simulink model "sys1"  (R2023b)
settings: Solver=VariableStepAuto  StartTime=0.0  StopTime=30e-3  RelTol=1e-3
InitFcn:
  | fs = 100e6;
  | ts = 1 / fs;
values from neighbouring files (symbols this model uses):
  c = 3e8    (= 300000000)    [init_param.m]
  H_az1 = zeros(numSamples,numPulses)    [init_param.m]
  H_az2 = zeros(numSamples,numPulses)    [init_param.m]
  H_ref = fft(conj(fliplr(txChirp)), numSamples)    [init_param.m]
  rawData = rawData + 0.01 * (randn(size(rawData)) + 1j * randn(size(rawData)))    [init_param.m]
  x1 = zeros(size(rawData))    [main.m]
  x2 = zeros(size(x1))    [main.m]
  x3 = zeros(size(x2))    [main.m]
  x4 = zeros(size(x3))    [main.m]
  x5 = zeros(size(x4))    [main.m]
  x6 = zeros(size(x5))    [main.m]
  xx4 = zeros(size(xx3))    [main.m]
  xx5 = zeros(size(xx4))    [main.m]
  xx6 = zeros(size(xx5))    [main.m]
undefined symbols (not defined in the file or in its folder): ffva1156, w2, w3, w4, w5, w6, w7, w8, w9, ww2, ww3, ww4, ww5, ww6, ww7, ww8, ww9, xcku095
libraries: hdlBasic x917, hdlDSPIP x18, dspsrcs4 x12, vmcUtilities x1
(part 1 of 9)
settings Model: Creator=abbas  LastModifiedBy=87544

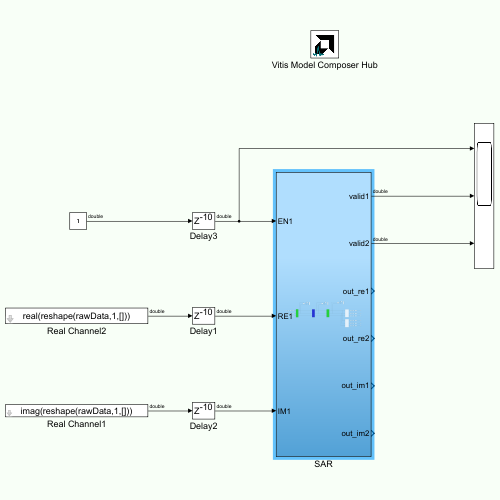
[thumbnail: Simulink's stored preview of the top-level diagram]
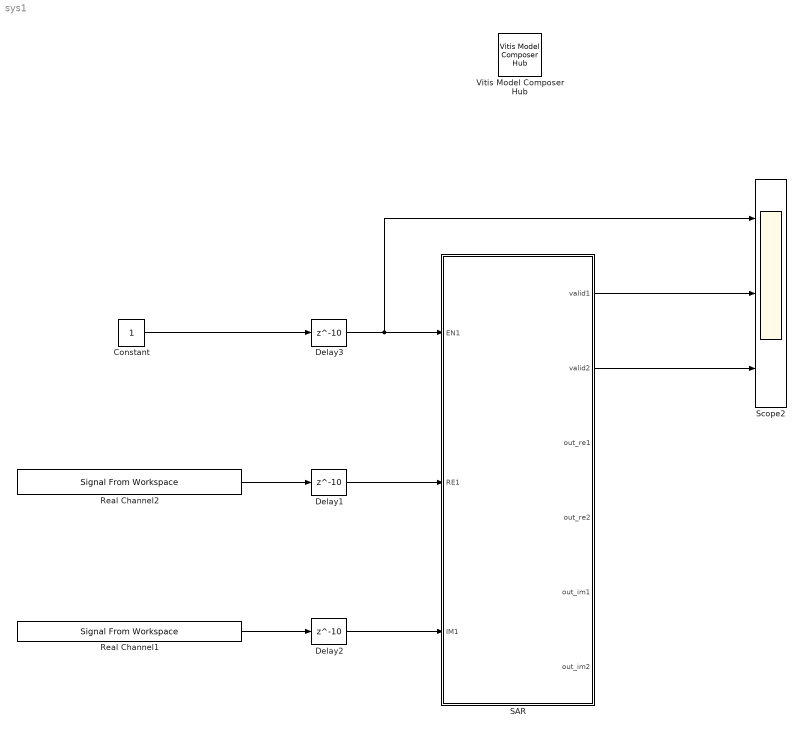
== system sys1 ==
  Constant : Constant
  Delay1 : Delay  DelayLength=10  InitialCondition=0  UseCircularBuffer=on
  Delay2 : Delay  DelayLength=10  InitialCondition=0  UseCircularBuffer=on
  Delay3 : Delay  DelayLength=10  InitialCondition=0  UseCircularBuffer=on
  Real Channel1 : dspsrcs4/Signal From Workspace  X=imag(reshape(rawData,1,[]))  Ts=ts  nsamps=1  OutputAfterFinalValue=Cyclic repetition  ignoreOrWarnInputAndFrameLengths=off  OutputFrames=on
  Real Channel2 : dspsrcs4/Signal From Workspace  X=real(reshape(rawData,1,[]))  Ts=ts  nsamps=1  OutputAfterFinalValue=Cyclic repetition  ignoreOrWarnInputAndFrameLengths=off  OutputFrames=on
  SAR : Subsystem
  Scope2 : Scope  NumInputPorts=3
  Vitis Model Composer Hub : vmcUtilities/Vitis Model Composer Hub  Tag=genX  CodeGeneration=off  SubsystemName=sar_sys8  TargetDirectory=./code  ExportType=System Generator  IpVendor=xilinx.com  IpLibrary=hls  IpVersion=1.0  IpHWLanguage=Verilog  AieCompilerOptions={}  AieSimulatorOptions={}  CreateTestbench=off  TestbenchStackSize=10  RunRtlSim=off  RunCSim=off  RunAieSim=off  AieSimTimeout=50000  RunAieSimProfiling=off  LaunchVitisAnalyzer=off  PlotOutput=off  RunX86Sim=off  X86SimTimeout=10  GenHwImage=off  GenLibadfXo=off  PlatformType=Not Specified  HwSystemType=Baremetal  HwValidationTarget=hw  ProjDevice=xcku095-ffva1156-1-c  ProjDevicePart=xcku095-ffva1156-1-c  AIEType=None  SamplePeriod=-1  ClockFrequency=200  DataPathParallelism=1  xilinxfamily=kintexu  part=xcku095  speed=-1-c  package=ffva1156  directory=C:/Users/87544/Desktop/Low-Latency SAR Processing/mat/netlist\ip\sar_sys8\src  testbench=off  incr_netlist=off  synthesis_tool=Vivado  clock_wrapper=Clock Enables  dbl_ovrd=According to Block Masks  dcm_input_clock_period=10  sysclk_period=10  simulink_period=10e-9  eval_field=0  IPInfoJsonString="{\"HDLSubsystem\":{\"SubsystemName\":\"SAR\",\"IPName\":\"SAR\",\"IPLibrary\":\"VMC\",\"IPVendor\":\"User Company\",\"IPVersion\":\"1.0\",\"TargetDirectory\":\"C:/Users/87544/Desktop/SAR/netlist\",\"SubsystemDir\":\"C:/Users/87544/Desktop/SAR/netlist\\\\ip\\\\SAR\"}}"  LogFileName=''  NThreads=4
  wires:
  Delay3/1 -> Scope2/1, SAR/1(EN1)
  Real Channel2/1 -> Delay1/1
  Constant/1 -> Delay3/1
  Delay2/1 -> SAR/3(IM1)
  Real Channel1/1 -> Delay2/1
  Delay1/1 -> SAR/2(RE1)
  SAR/1(valid1) -> Scope2/2
  SAR/2(valid2) -> Scope2/3

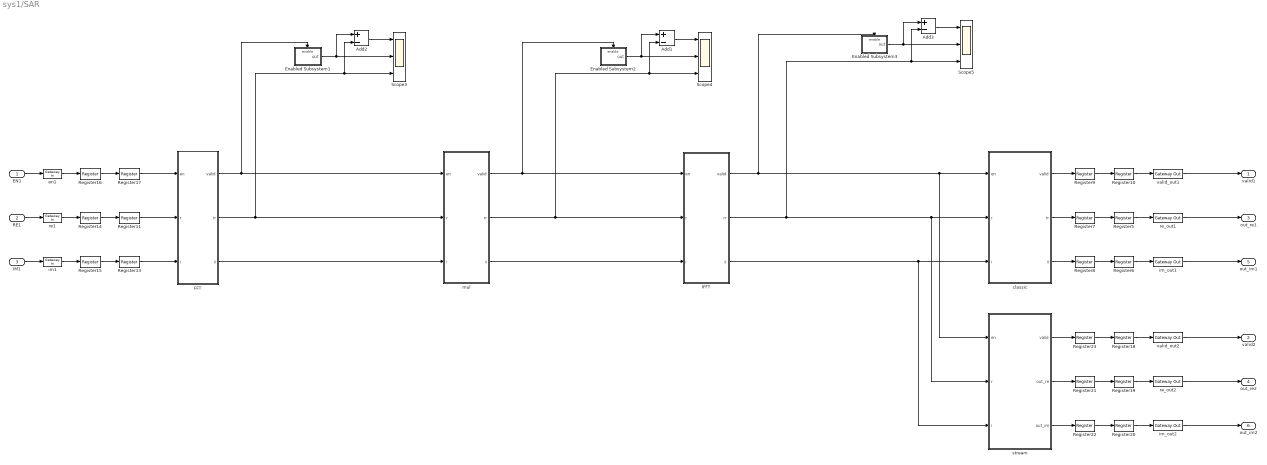
== system sys1/SAR ==
  EN1 : Inport
  RE1 : Inport  Port=2
  IM1 : Inport  Port=3
  Add1 : Sum  Inputs=+-
  Add2 : Sum  Inputs=+-
  Add3 : Sum  Inputs=+-
  Enabled Subsystem1 : Subsystem  TreatAsAtomicUnit=on
  Enabled Subsystem2 : Subsystem  TreatAsAtomicUnit=on
  Enabled Subsystem3 : Subsystem  TreatAsAtomicUnit=on
  FFT : Subsystem
  IFFT : Subsystem
  Register{5..11,13..23} (18 alike) : hdlBasic/Register  init=0  rst=off  en=off  XmcBlockStatus=1  maskContainerNames=tabcontainer1  block_type=register  block_config=sysgen:Register_config
  Scope3 : Scope  NumInputPorts=3
  Scope4 : Scope  NumInputPorts=3
  Scope5 : Scope  NumInputPorts=3
  classic : Subsystem
  en1 : hdlBasic/Gateway In  gui_display_data_type=Boolean  arith_type=Boolean  n_bits=16  bin_pt=15  preci_type=Single  exp_width=8  frac_width=24  rows=1  columns=1  quantization="Round  (unbiased: +/- Inf)"  overflow=Saturate  period=ts  UseAsADC=off  ADCChannel='1'  interface=None  automatic_assignment=on  address_offset=hex2dec('00')  intf_name=''  intf_description=''  default_value=0  timing_constraint=None  locs_specified=off  LOCs={}  io_standard={}  inherit_from_input=off  hdl_port=on  XmcBlockStatus=1  maskContainerNames=group4  block_type=gatewayin  block_config=sysgen:gateway_in_config  block_width_w=590  block_height_w=620  block_width=640  block_height=850
  im1 : hdlBasic/Gateway In  gui_display_data_type=Fixed-point  arith_type=Signed (2's comp)  n_bits=16  bin_pt=15  preci_type=Single  exp_width=8  frac_width=24  rows=1  columns=1  quantization="Round  (unbiased: +/- Inf)"  overflow=Saturate  period=ts  UseAsADC=off  ADCChannel='1'  interface=None  automatic_assignment=on  address_offset=hex2dec('00')  intf_name=''  intf_description=''  default_value=0  timing_constraint=None  locs_specified=off  LOCs={}  io_standard={}  inherit_from_input=off  hdl_port=on  XmcBlockStatus=1  maskContainerNames=group4  block_type=gatewayin  block_config=sysgen:gateway_in_config  block_width_w=590  block_height_w=620  block_width=640  block_height=850
  im_out1 : hdlBasic/Gateway Out  inherit_from_input=off  hdl_port=on  rows=1  columns=1  UseAsDAC=off  DACChannel='1'  interface=None  automatic_assignment=on  address_offset=hex2dec('00')  intf_name=''  intf_description=''  timing_constraint=None  locs_specified=off  LOCs={}  io_standard={}  XmcBlockStatus=1  maskContainerNames=group4  block_type=gatewayout  block_config=sysgen:gateway_out_config  block_width_w=590  block_height_w=620  block_width=620  block_height=750
  im_out2 : hdlBasic/Gateway Out  inherit_from_input=off  hdl_port=on  rows=1  columns=1  UseAsDAC=off  DACChannel='1'  interface=None  automatic_assignment=on  address_offset=hex2dec('00')  intf_name=''  intf_description=''  timing_constraint=None  locs_specified=off  LOCs={}  io_standard={}  XmcBlockStatus=1  maskContainerNames=group4  block_type=gatewayout  block_config=sysgen:gateway_out_config  block_width_w=590  block_height_w=620  block_width=620  block_height=750
  mul : Subsystem
  re1 : hdlBasic/Gateway In  gui_display_data_type=Fixed-point  arith_type=Signed (2's comp)  n_bits=16  bin_pt=15  preci_type=Single  exp_width=8  frac_width=24  rows=1  columns=1  quantization="Round  (unbiased: +/- Inf)"  overflow=Saturate  period=ts  UseAsADC=off  ADCChannel='1'  interface=None  automatic_assignment=on  address_offset=hex2dec('00')  intf_name=''  intf_description=''  default_value=0  timing_constraint=None  locs_specified=off  LOCs={}  io_standard={}  inherit_from_input=off  hdl_port=on  XmcBlockStatus=1  maskContainerNames=group4  block_type=gatewayin  block_config=sysgen:gateway_in_config  block_width_w=590  block_height_w=620  block_width=640  block_height=850
  re_out1 : hdlBasic/Gateway Out  inherit_from_input=off  hdl_port=on  rows=1  columns=1  UseAsDAC=off  DACChannel='1'  interface=None  automatic_assignment=on  address_offset=hex2dec('00')  intf_name=''  intf_description=''  timing_constraint=None  locs_specified=off  LOCs={}  io_standard={}  XmcBlockStatus=1  maskContainerNames=group4  block_type=gatewayout  block_config=sysgen:gateway_out_config  block_width_w=590  block_height_w=620  block_width=620  block_height=750
  re_out2 : hdlBasic/Gateway Out  inherit_from_input=off  hdl_port=on  rows=1  columns=1  UseAsDAC=off  DACChannel='1'  interface=None  automatic_assignment=on  address_offset=hex2dec('00')  intf_name=''  intf_description=''  timing_constraint=None  locs_specified=off  LOCs={}  io_standard={}  XmcBlockStatus=1  maskContainerNames=group4  block_type=gatewayout  block_config=sysgen:gateway_out_config  block_width_w=590  block_height_w=620  block_width=620  block_height=750
  stream : Subsystem
  valid_out1 : hdlBasic/Gateway Out  inherit_from_input=off  hdl_port=on  rows=1  columns=1  UseAsDAC=off  DACChannel='1'  interface=None  automatic_assignment=on  address_offset=hex2dec('00')  intf_name=''  intf_description=''  timing_constraint=None  locs_specified=off  LOCs={}  io_standard={}  XmcBlockStatus=1  maskContainerNames=group4  block_type=gatewayout  block_config=sysgen:gateway_out_config  block_width_w=590  block_height_w=620  block_width=620  block_height=750
  valid_out2 : hdlBasic/Gateway Out  inherit_from_input=off  hdl_port=on  rows=1  columns=1  UseAsDAC=off  DACChannel='1'  interface=None  automatic_assignment=on  address_offset=hex2dec('00')  intf_name=''  intf_description=''  timing_constraint=None  locs_specified=off  LOCs={}  io_standard={}  XmcBlockStatus=1  maskContainerNames=group4  block_type=gatewayout  block_config=sysgen:gateway_out_config  block_width_w=590  block_height_w=620  block_width=620  block_height=750
  valid1 : Outport
  valid2 : Outport  Port=2
  out_re1 : Outport  Port=3
  out_re2 : Outport  Port=4
  out_im1 : Outport  Port=5
  out_im2 : Outport  Port=6
  wires:
  EN1/1 -> en1/1
  IM1/1 -> im1/1
  RE1/1 -> re1/1
  Register22/1 -> Register20/1
  classic/3(ii) -> Register8/1
  Register9/1 -> Register10/1
  en1/1 -> Register16/1
  re1/1 -> Register14/1
  im1/1 -> Register15/1
  Register19/1 -> re_out2/1
  Register16/1 -> Register17/1
  Register20/1 -> im_out2/1
  Register14/1 -> Register11/1
  Register15/1 -> Register13/1
  stream/2(out_re) -> Register21/1
  stream/1(valid) -> Register23/1
  stream/3(out_im) -> Register22/1
  Register18/1 -> valid_out2/1
  classic/2(rr) -> Register7/1
  classic/1(valid) -> Register9/1
  Register23/1 -> Register18/1
  Register21/1 -> Register19/1
  Register7/1 -> Register5/1
  Register8/1 -> Register6/1
  Register10/1 -> valid_out1/1
  Register5/1 -> re_out1/1
  Register6/1 -> im_out1/1
  valid_out2/1 -> valid2/1
  re_out2/1 -> out_re2/1
  im_out2/1 -> out_im2/1
  valid_out1/1 -> valid1/1
  re_out1/1 -> out_re1/1
  im_out1/1 -> out_im1/1
  FFT/2(rr) -> mul/2(r), Add2/2, Scope3/3
  mul/2(rr) -> Scope4/3, Add1/2, IFFT/2(r)
  Register11/1 -> FFT/2(r)
  FFT/1(valid) -> mul/1(en), Enabled Subsystem1/Enable
  Add3/1 -> Scope5/1
  Add1/1 -> Scope4/1
  Enabled Subsystem3/1(out) -> Add3/1, Scope5/2
  IFFT/1(valid) -> stream/1(en), classic/1(en), Enabled Subsystem3/Enable
  mul/1(valid) -> IFFT/1(en), Enabled Subsystem2/Enable
  Register13/1 -> FFT/3(i)
  Enabled Subsystem2/1(out) -> Scope4/2, Add1/1
  Enabled Subsystem1/1(out) -> Add2/1, Scope3/2
  Register17/1 -> FFT/1(en)
  Add2/1 -> Scope3/1
  mul/3(ii) -> IFFT/3(i)
  FFT/3(ii) -> mul/3(i)
  IFFT/2(rr) -> stream/2(r), classic/2(r), Add3/2, Scope5/3
  IFFT/3(ii) -> stream/3(i), classic/3(i)

== system sys1/SAR/Enabled Subsystem1 ==
  Enable : EnablePort
  Real Channel4 : dspsrcs4/Signal From Workspace  X=real(reshape(x1,1,[]))/2^6  Ts=ts  nsamps=1  OutputAfterFinalValue=Cyclic repetition  ignoreOrWarnInputAndFrameLengths=off  OutputFrames=on
  out : Outport
  wires:
  Real Channel4/1 -> out/1

== system sys1/SAR/Enabled Subsystem2 ==
  Enable : EnablePort
  Real Channel4 : dspsrcs4/Signal From Workspace  X=real(reshape(x2,1,[]))*2^-10  Ts=ts  nsamps=1  OutputAfterFinalValue=Cyclic repetition  ignoreOrWarnInputAndFrameLengths=off  OutputFrames=on
  out : Outport
  wires:
  Real Channel4/1 -> out/1

== system sys1/SAR/Enabled Subsystem3 ==
  Enable : EnablePort
  Real Channel4 : dspsrcs4/Signal From Workspace  X=real(reshape(x3,1,[]))*2^-7  Ts=ts  nsamps=1  OutputAfterFinalValue=Cyclic repetition  ignoreOrWarnInputAndFrameLengths=off  OutputFrames=on
  out : Outport
  wires:
  Real Channel4/1 -> out/1

== system sys1/SAR/FFT ==
  en : Inport
  r : Inport  Port=2
  i : Inport  Port=3
  Constant1 : hdlBasic/Constant  const=1.0  gui_display_data_type=Boolean  arith_type=Boolean  n_bits=16  bin_pt=14  preci_type=Single  exp_width=8  frac_width=24  explicit_period=on  period=ts  XmcBlockStatus=1  maskContainerNames=tabcontainer1  block_type=constant  block_config=sysgen:Constant_config
  FFT : hdlBasic/FFT  transform_length=1024  scale_result_by_fft_length=on  bit_reversed_order=on  optimizegoal=Performance  start_frame=on  simulation_type=fast_sim  simulation_model=sysgen:ForwardFFT_Macro  latency=1  XmcBlockStatus=1  maskContainerNames=group1  block_type=xfft_forward  block_config=sysgen:FFTMacro_config
  Register5 : hdlBasic/Register  init=0  rst=off  en=off  XmcBlockStatus=1  maskContainerNames=tabcontainer1  block_type=register  block_config=sysgen:Register_config
  Register6 : hdlBasic/Register  init=0  rst=off  en=off  XmcBlockStatus=1  maskContainerNames=tabcontainer1  block_type=register  block_config=sysgen:Register_config
  Register7 : hdlBasic/Register  init=0  rst=off  en=on  XmcBlockStatus=1  maskContainerNames=tabcontainer1  block_type=register  block_config=sysgen:Register_config
  Shift1 : hdlBasic/Shift  shift_dir=Left  shift_bits=5  en=off  latency=0  precision=User Defined  arith_type="Signed  (2's comp)"  n_bits=16  bin_pt=15  quantization="Round  (unbiased: +/- Inf)"  overflow=Flag as error  XmcBlockStatus=1  maskContainerNames=group2  block_type=shift  block_config=sysgen:Shift_config
  Shift3 : hdlBasic/Shift  shift_dir=Left  shift_bits=5  en=off  latency=0  precision=User Defined  arith_type="Signed  (2's comp)"  n_bits=16  bin_pt=15  quantization="Round  (unbiased: +/- Inf)"  overflow=Flag as error  XmcBlockStatus=1  maskContainerNames=group2  block_type=shift  block_config=sysgen:Shift_config
  valid : Outport
  rr : Outport  Port=2
  ii : Outport  Port=3
  wires:
  Register6/1 -> Shift1/1
  Register5/1 -> Shift3/1
  i/1 -> FFT/2
  FFT/1 -> Register5/1
  en/1 -> FFT/3
  r/1 -> FFT/1
  FFT/3 -> Register7/2
  Constant1/1 -> Register7/1
  FFT/2 -> Register6/1
  Shift1/1 -> ii/1
  Register7/1 -> valid/1
  Shift3/1 -> rr/1

== system sys1/SAR/IFFT ==
  en : Inport
  r : Inport  Port=2
  i : Inport  Port=3
  Constant1 : hdlBasic/Constant  const=1  gui_display_data_type=Boolean  arith_type=Boolean  n_bits=16  bin_pt=14  preci_type=Single  exp_width=8  frac_width=24  explicit_period=on  period=ts  XmcBlockStatus=1  maskContainerNames=tabcontainer1  block_type=constant  block_config=sysgen:Constant_config
  Inverse FFT : hdlBasic/Inverse FFT  transform_length=1024  scale_result_by_fft_length=on  bit_reversed_order=on  optimizegoal=Performance  start_frame=on  simulation_type=fast_sim  simulation_model=sysgen:InverseFFT_Macro  latency=1  XmcBlockStatus=1  maskContainerNames=group1  block_type=xfft_inverse  block_config=sysgen:Inverse_FFTMacro_config
  Register1 : hdlBasic/Register  init=0  rst=off  en=off  XmcBlockStatus=1  maskContainerNames=tabcontainer1  block_type=register  block_config=sysgen:Register_config
  Register2 : hdlBasic/Register  init=0  rst=off  en=on  XmcBlockStatus=1  maskContainerNames=tabcontainer1  block_type=register  block_config=sysgen:Register_config
  Register5 : hdlBasic/Register  init=0  rst=off  en=off  XmcBlockStatus=1  maskContainerNames=tabcontainer1  block_type=register  block_config=sysgen:Register_config
  Shift1 : hdlBasic/Shift  shift_dir=Left  shift_bits=4  en=off  latency=0  precision=User Defined  arith_type="Signed  (2's comp)"  n_bits=16  bin_pt=15  quantization="Round  (unbiased: +/- Inf)"  overflow=Flag as error  XmcBlockStatus=1  maskContainerNames=group2  block_type=shift  block_config=sysgen:Shift_config
  Shift2 : hdlBasic/Shift  shift_dir=Left  shift_bits=4  en=off  latency=0  precision=User Defined  arith_type="Signed  (2's comp)"  n_bits=16  bin_pt=15  quantization="Round  (unbiased: +/- Inf)"  overflow=Flag as error  XmcBlockStatus=1  maskContainerNames=group2  block_type=shift  block_config=sysgen:Shift_config
  valid : Outport
  rr : Outport  Port=2
  ii : Outport  Port=3
  wires:
  Register2/1 -> valid/1
  Inverse FFT/3 -> Register2/2
  Constant1/1 -> Register2/1
  Inverse FFT/2 -> Register1/1
  Inverse FFT/1 -> Register5/1
  en/1 -> Inverse FFT/3
  i/1 -> Inverse FFT/2
  r/1 -> Inverse FFT/1
  Register5/1 -> Shift1/1
  Register1/1 -> Shift2/1
  Shift1/1 -> rr/1
  Shift2/1 -> ii/1

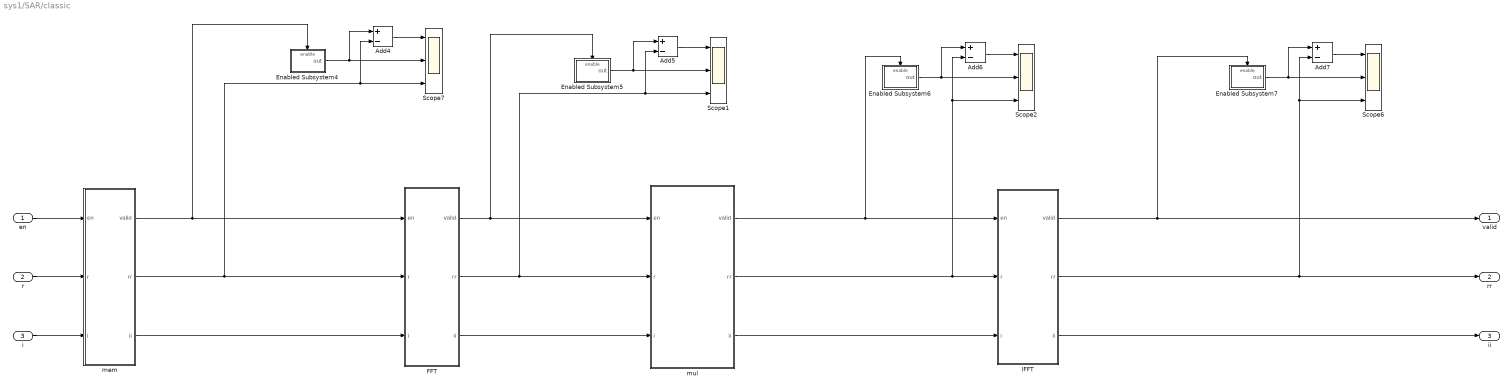
== system sys1/SAR/classic ==
  en : Inport
  r : Inport  Port=2
  i : Inport  Port=3
  Add{4..7} (4 alike) : Sum  Inputs=+-
  Enabled Subsystem4 : Subsystem  TreatAsAtomicUnit=on
  Enabled Subsystem5 : Subsystem  TreatAsAtomicUnit=on
  Enabled Subsystem6 : Subsystem  TreatAsAtomicUnit=on
  Enabled Subsystem7 : Subsystem  TreatAsAtomicUnit=on
  FFT : Subsystem
  IFFT : Subsystem
  Scope{1..2,6..7} (4 alike) : Scope  NumInputPorts=3
  mem : Subsystem
  mul : Subsystem
      mask Display: %%
  valid : Outport
  rr : Outport  Port=2
  ii : Outport  Port=3
  wires:
  Enabled Subsystem6/1(out) -> Scope2/2, Add6/1
  mem/2(rr) -> Scope7/3, Add4/2, FFT/2(r)
  FFT/3(ii) -> mul/3(i)
  mul/1(valid) -> IFFT/1(en), Enabled Subsystem6/Enable
  mul/2(rr) -> IFFT/2(r), Scope2/3, Add6/2
  mul/3(ii) -> IFFT/3(i)
  Add4/1 -> Scope7/1
  FFT/2(rr) -> mul/2(r), Add5/2, Scope1/3
  mem/1(valid) -> Enabled Subsystem4/Enable, FFT/1(en)
  IFFT/2(rr) -> rr/1, Add7/2, Scope6/3
  r/1 -> mem/2(r)
  FFT/1(valid) -> mul/1(en), Enabled Subsystem5/Enable
  IFFT/3(ii) -> ii/1
  mem/3(ii) -> FFT/3(i)
  Add5/1 -> Scope1/1
  i/1 -> mem/3(i)
  Enabled Subsystem4/1(out) -> Scope7/2, Add4/1
  Enabled Subsystem5/1(out) -> Add5/1, Scope1/2
  Add6/1 -> Scope2/1
  Enabled Subsystem7/1(out) -> Add7/1, Scope6/2
  IFFT/1(valid) -> valid/1, Enabled Subsystem7/Enable
  Add7/1 -> Scope6/1
  en/1 -> mem/1(en)

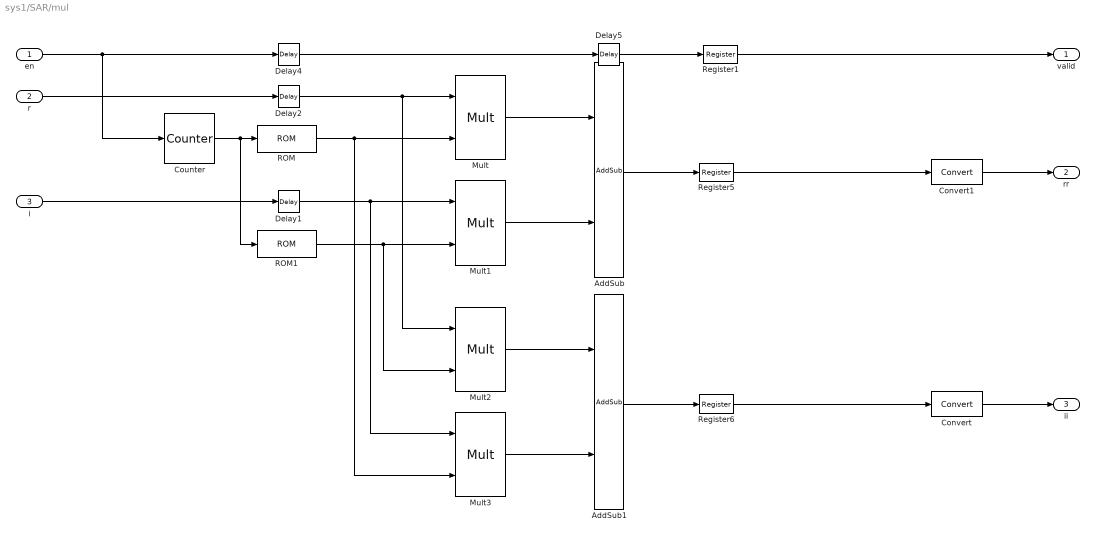
== system sys1/SAR/mul ==
  en : Inport
  r : Inport  Port=2
  i : Inport  Port=3
  AddSub : hdlBasic/AddSub  mode=Subtraction  use_carryin=off  use_carryout=off  en=off  latency=1  precision=Full  arith_type=Unsigned  n_bits=16  bin_pt=14  quantization=Truncate  overflow=Wrap  use_behavioral_HDL=off  hw_selection=Fabric  pipelined=off  XmcBlockStatus=1  maskContainerNames=tabcontainer1  block_type=addsub  block_config=sysgen:Addsub_config
  AddSub1 : hdlBasic/AddSub  mode=Addition  use_carryin=off  use_carryout=off  en=off  latency=1  precision=Full  arith_type=Unsigned  n_bits=16  bin_pt=14  quantization=Truncate  overflow=Wrap  use_behavioral_HDL=off  hw_selection=Fabric  pipelined=off  XmcBlockStatus=1  maskContainerNames=tabcontainer1  block_type=addsub  block_config=sysgen:Addsub_config
  Convert : hdlBasic/Convert  gui_display_data_type=Fixed-point  arith_type=Signed (2's comp)  n_bits=16  bin_pt=15  float_type=Single  exp_bits=8  fraction_bits=24  quantization="Round  (unbiased: +/- Inf)"  overflow=Saturate  en=off  latency=0  pipeline=off  XmcBlockStatus=1  maskContainerNames=group2  block_type=convert  block_config=sysgen:Convert_config  block_width=595  block_height=885
  Convert1 : hdlBasic/Convert  gui_display_data_type=Fixed-point  arith_type=Signed (2's comp)  n_bits=16  bin_pt=15  float_type=Single  exp_bits=8  fraction_bits=24  quantization="Round  (unbiased: +/- Inf)"  overflow=Saturate  en=off  latency=0  pipeline=off  XmcBlockStatus=1  maskContainerNames=group2  block_type=convert  block_config=sysgen:Convert_config  block_width=595  block_height=885
  Counter : hdlBasic/Counter  cnt_type=Free running  cnt_to=Inf  operation=Up  start_count=0  cnt_by_val=1  arith_type=Unsigned  n_bits=10  bin_pt=0  load_pin=off  rst=off  en=on  explicit_period=Explicit  period=ts  use_behavioral_HDL=off  implementation=Fabric  XmcBlockStatus=1  maskContainerNames=group1  block_type=counter  block_config=sysgen:Counter_config  block_width=531  block_height=1023
  Delay1 : hdlBasic/Delay  rst=off  en=off  latency=1  reg_retiming=off  XmcBlockStatus=1  maskContainerNames=group1  block_type=delay  block_config=sysgen:Delay_config
  Delay2 : hdlBasic/Delay  rst=off  en=off  latency=1  reg_retiming=off  XmcBlockStatus=1  maskContainerNames=group1  block_type=delay  block_config=sysgen:Delay_config
  Delay4 : hdlBasic/Delay  rst=off  en=off  latency=1  reg_retiming=off  XmcBlockStatus=1  maskContainerNames=group1  block_type=delay  block_config=sysgen:Delay_config
  Delay5 : hdlBasic/Delay  rst=off  en=off  latency=4  reg_retiming=off  XmcBlockStatus=1  maskContainerNames=group1  block_type=delay  block_config=sysgen:Delay_config
  Mult{,1..3} (4 alike) : hdlBasic/Mult  precision=Full  arith_type="Signed  (2's comp)"  n_bits=16  bin_pt=14  quantization=Truncate  overflow=Wrap  en=off  latency=3  use_behavioral_HDL=off  opt=Speed  use_embedded=on  optimum_pipeline=off  pipeline=on  use_rpm=on  placement_style=Triangular  XmcBlockStatus=1  maskContainerNames=group1  block_type=mult  block_config=sysgen:Mult_config  block_width=598  block_height=876
  ROM : hdlBasic/ROM  depth=1024  initVector=double(real(H_ref/16))  distributed_mem=Block RAM  rst=off  init_reg=0  en=off  latency=1  gui_display_data_type=Fixed-point  arith_type="Signed  (2's comp)"  n_bits=16  bin_pt=15  preci_type=Single  exp_width=8  frac_width=24  optimize=Area  use_rpm=on  simulation_type=fast_sim  XmcBlockStatus=1  maskContainerNames=tabcontainer1  block_type=sprom  block_config=sysgen:SPROM_config
  ROM1 : hdlBasic/ROM  depth=1024  initVector=double(imag(H_ref/16))  distributed_mem=Block RAM  rst=off  init_reg=0  en=off  latency=1  gui_display_data_type=Fixed-point  arith_type="Signed  (2's comp)"  n_bits=16  bin_pt=15  preci_type=Single  exp_width=8  frac_width=24  optimize=Area  use_rpm=on  simulation_type=fast_sim  XmcBlockStatus=1  maskContainerNames=tabcontainer1  block_type=sprom  block_config=sysgen:SPROM_config
  Register1 : hdlBasic/Register  init=0  rst=off  en=off  XmcBlockStatus=1  maskContainerNames=tabcontainer1  block_type=register  block_config=sysgen:Register_config
  Register5 : hdlBasic/Register  init=0  rst=off  en=off  XmcBlockStatus=1  maskContainerNames=tabcontainer1  block_type=register  block_config=sysgen:Register_config
  Register6 : hdlBasic/Register  init=0  rst=off  en=off  XmcBlockStatus=1  maskContainerNames=tabcontainer1  block_type=register  block_config=sysgen:Register_config
  valid : Outport
  rr : Outport  Port=2
  ii : Outport  Port=3
  wires:
  ROM1/1 -> Mult1/2, Mult2/2
  Delay2/1 -> Mult/1, Mult2/1
  Delay1/1 -> Mult3/1, Mult1/1
  ROM/1 -> Mult/2, Mult3/2
  Register1/1 -> valid/1
  AddSub1/1 -> Register6/1
  Mult3/1 -> AddSub1/2
  Mult2/1 -> AddSub1/1
  Delay5/1 -> Register1/1
  Mult1/1 -> AddSub/2
  Mult/1 -> AddSub/1
  AddSub/1 -> Register5/1
  Convert1/1 -> rr/1
  Convert/1 -> ii/1
  Delay4/1 -> Delay5/1
  Counter/1 -> ROM/1, ROM1/1
  r/1 -> Delay2/1
  en/1 -> Counter/1, Delay4/1
  i/1 -> Delay1/1
  Register5/1 -> Convert1/1
  Register6/1 -> Convert/1

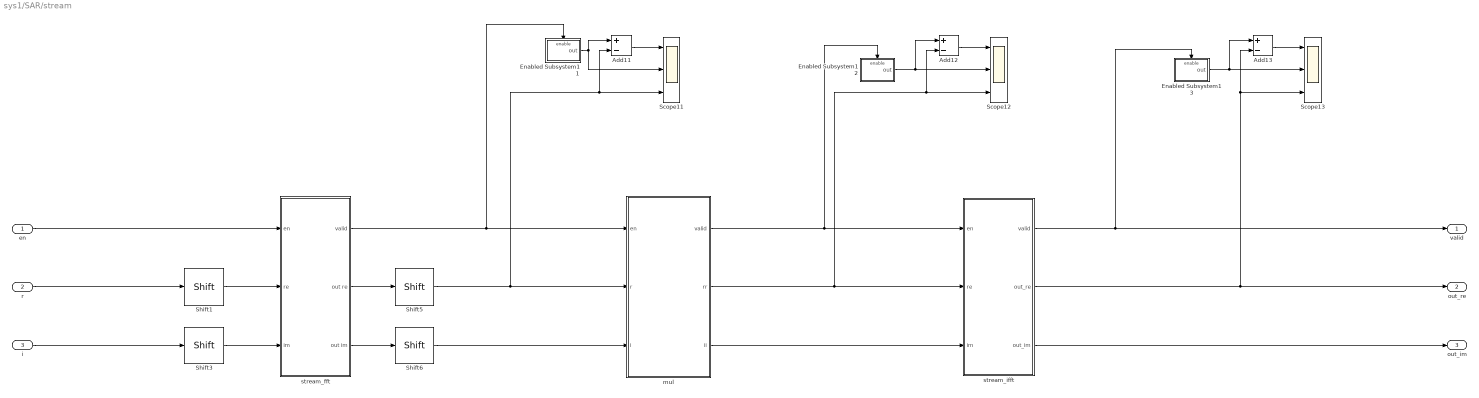
== system sys1/SAR/stream ==
  en : Inport
  r : Inport  Port=2
  i : Inport  Port=3
  Add11 : Sum  Inputs=+-
  Add12 : Sum  Inputs=+-
  Add13 : Sum  Inputs=+-
  Enabled Subsystem11 : Subsystem  TreatAsAtomicUnit=on
  Enabled Subsystem12 : Subsystem  TreatAsAtomicUnit=on
  Enabled Subsystem13 : Subsystem  TreatAsAtomicUnit=on
  Scope11 : Scope  NumInputPorts=3
  Scope12 : Scope  NumInputPorts=3
  Scope13 : Scope  NumInputPorts=3
  Shift1 : hdlBasic/Shift  shift_dir=Right  shift_bits=3  en=off  latency=0  precision=User Defined  arith_type="Signed  (2's comp)"  n_bits=16  bin_pt=15  quantization="Round  (unbiased: +/- Inf)"  overflow=Flag as error  XmcBlockStatus=1  maskContainerNames=group2  block_type=shift  block_config=sysgen:Shift_config
  Shift3 : hdlBasic/Shift  shift_dir=Right  shift_bits=3  en=off  latency=0  precision=User Defined  arith_type="Signed  (2's comp)"  n_bits=16  bin_pt=15  quantization="Round  (unbiased: +/- Inf)"  overflow=Flag as error  XmcBlockStatus=1  maskContainerNames=group2  block_type=shift  block_config=sysgen:Shift_config
  Shift5 : hdlBasic/Shift  shift_dir=Left  shift_bits=6  en=off  latency=0  precision=User Defined  arith_type="Signed  (2's comp)"  n_bits=16  bin_pt=15  quantization="Round  (unbiased: +/- Inf)"  overflow=Flag as error  XmcBlockStatus=1  maskContainerNames=group2  block_type=shift  block_config=sysgen:Shift_config
  Shift6 : hdlBasic/Shift  shift_dir=Left  shift_bits=6  en=off  latency=0  precision=User Defined  arith_type="Signed  (2's comp)"  n_bits=16  bin_pt=15  quantization="Round  (unbiased: +/- Inf)"  overflow=Flag as error  XmcBlockStatus=1  maskContainerNames=group2  block_type=shift  block_config=sysgen:Shift_config
  mul : Subsystem
  stream_fft : Subsystem
  stream_ifft : Subsystem
  valid : Outport
  out_re : Outport  Port=2
  out_im : Outport  Port=3
  wires:
  Enabled Subsystem12/1(out) -> Scope12/2, Add12/1
  Enabled Subsystem11/1(out) -> Scope11/2, Add11/1
  stream_fft/2(out re) -> Shift5/1
  Add12/1 -> Scope12/1
  Add11/1 -> Scope11/1
  r/1 -> Shift1/1
  stream_fft/1(valid) -> mul/1(en), Enabled Subsystem11/Enable
  stream_ifft/1(valid) -> valid/1, Enabled Subsystem13/Enable
  Add13/1 -> Scope13/1
  i/1 -> Shift3/1
  stream_fft/3(out im) -> Shift6/1
  mul/1(valid) -> stream_ifft/1(en), Enabled Subsystem12/Enable
  stream_ifft/2(out_re) -> out_re/1, Add13/2, Scope13/3
  Enabled Subsystem13/1(out) -> Add13/1, Scope13/2
  stream_ifft/3(out_im) -> out_im/1
  en/1 -> stream_fft/1(en)
  Shift1/1 -> stream_fft/2(re)
  Shift3/1 -> stream_fft/3(im)
  Shift5/1 -> mul/2(r), Add11/2, Scope11/3
  Shift6/1 -> mul/3(i)
  mul/2(rr) -> stream_ifft/2(re), Scope12/3, Add12/2
  mul/3(ii) -> stream_ifft/3(im)

== system sys1/SAR/classic/Enabled Subsystem4 ==
  Enable : EnablePort
  Real Channel4 : dspsrcs4/Signal From Workspace  X=real(reshape(x3',1,[]))*2^-7  Ts=ts  nsamps=1  OutputAfterFinalValue=Cyclic repetition  ignoreOrWarnInputAndFrameLengths=off  OutputFrames=on
  out : Outport
  wires:
  Real Channel4/1 -> out/1

== system sys1/SAR/classic/Enabled Subsystem5 ==
  Enable : EnablePort
  Real Channel4 : dspsrcs4/Signal From Workspace  X=real(reshape(x4',1,[]))*2^-13  Ts=ts  nsamps=1  OutputAfterFinalValue=Cyclic repetition  ignoreOrWarnInputAndFrameLengths=off  OutputFrames=on
  out : Outport
  wires:
  Real Channel4/1 -> out/1

== system sys1/SAR/classic/Enabled Subsystem6 ==
  Enable : EnablePort
  Real Channel4 : dspsrcs4/Signal From Workspace  X=real(reshape(x5',1,[]))*2^-13  Ts=ts  nsamps=1  OutputAfterFinalValue=Cyclic repetition  ignoreOrWarnInputAndFrameLengths=off  OutputFrames=on
  out : Outport
  wires:
  Real Channel4/1 -> out/1

== system sys1/SAR/classic/Enabled Subsystem7 ==
  Enable : EnablePort
  Real Channel4 : dspsrcs4/Signal From Workspace  X=real(reshape(x6',1,[]))*2^-8  Ts=ts  nsamps=1  OutputAfterFinalValue=Cyclic repetition  ignoreOrWarnInputAndFrameLengths=off  OutputFrames=on
  out : Outport
  wires:
  Real Channel4/1 -> out/1

== system sys1/SAR/classic/FFT ==
  en : Inport
  r : Inport  Port=2
  i : Inport  Port=3
  Constant1 : hdlBasic/Constant  const=1.0  gui_display_data_type=Boolean  arith_type=Boolean  n_bits=16  bin_pt=14  preci_type=Single  exp_width=8  frac_width=24  explicit_period=on  period=ts  XmcBlockStatus=1  maskContainerNames=tabcontainer1  block_type=constant  block_config=sysgen:Constant_config
  FFT : hdlBasic/FFT  transform_length=512  scale_result_by_fft_length=on  bit_reversed_order=on  optimizegoal=Performance  start_frame=on  simulation_type=fast_sim  simulation_model=sysgen:ForwardFFT_Macro  latency=1  XmcBlockStatus=1  maskContainerNames=group1  block_type=xfft_forward  block_config=sysgen:FFTMacro_config
  Register5 : hdlBasic/Register  init=0  rst=off  en=off  XmcBlockStatus=1  maskContainerNames=tabcontainer1  block_type=register  block_config=sysgen:Register_config
  Register6 : hdlBasic/Register  init=0  rst=off  en=off  XmcBlockStatus=1  maskContainerNames=tabcontainer1  block_type=register  block_config=sysgen:Register_config
  Register7 : hdlBasic/Register  init=0  rst=off  en=on  XmcBlockStatus=1  maskContainerNames=tabcontainer1  block_type=register  block_config=sysgen:Register_config
  Shift1 : hdlBasic/Shift  shift_dir=Left  shift_bits=4  en=off  latency=0  precision=User Defined  arith_type="Signed  (2's comp)"  n_bits=16  bin_pt=15  quantization="Round  (unbiased: +/- Inf)"  overflow=Flag as error  XmcBlockStatus=1  maskContainerNames=group2  block_type=shift  block_config=sysgen:Shift_config
  Shift2 : hdlBasic/Shift  shift_dir=Left  shift_bits=4  en=off  latency=0  precision=User Defined  arith_type="Signed  (2's comp)"  n_bits=16  bin_pt=15  quantization="Round  (unbiased: +/- Inf)"  overflow=Flag as error  XmcBlockStatus=1  maskContainerNames=group2  block_type=shift  block_config=sysgen:Shift_config
  valid : Outport
  rr : Outport  Port=2
  ii : Outport  Port=3
  wires:
  FFT/2 -> Register6/1
  Constant1/1 -> Register7/1
  FFT/3 -> Register7/2
  r/1 -> FFT/1
  en/1 -> FFT/3
  Register7/1 -> valid/1
  FFT/1 -> Register5/1
  i/1 -> FFT/2
  Register5/1 -> Shift1/1
  Register6/1 -> Shift2/1
  Shift1/1 -> rr/1
  Shift2/1 -> ii/1

== system sys1/SAR/classic/IFFT ==
  en : Inport
  r : Inport  Port=2
  i : Inport  Port=3
  Constant1 : hdlBasic/Constant  const=1  gui_display_data_type=Boolean  arith_type=Boolean  n_bits=16  bin_pt=14  preci_type=Single  exp_width=8  frac_width=24  explicit_period=on  period=ts  XmcBlockStatus=1  maskContainerNames=tabcontainer1  block_type=constant  block_config=sysgen:Constant_config
  Inverse FFT : hdlBasic/Inverse FFT  transform_length=512  scale_result_by_fft_length=on  bit_reversed_order=on  optimizegoal=Performance  start_frame=on  simulation_type=fast_sim  simulation_model=sysgen:InverseFFT_Macro  latency=1  XmcBlockStatus=1  maskContainerNames=group1  block_type=xfft_inverse  block_config=sysgen:Inverse_FFTMacro_config
  Register1 : hdlBasic/Register  init=0  rst=off  en=off  XmcBlockStatus=1  maskContainerNames=tabcontainer1  block_type=register  block_config=sysgen:Register_config
  Register2 : hdlBasic/Register  init=0  rst=off  en=on  XmcBlockStatus=1  maskContainerNames=tabcontainer1  block_type=register  block_config=sysgen:Register_config
  Register5 : hdlBasic/Register  init=0  rst=off  en=off  XmcBlockStatus=1  maskContainerNames=tabcontainer1  block_type=register  block_config=sysgen:Register_config
  Shift1 : hdlBasic/Shift  shift_dir=Left  shift_bits=6  en=off  latency=0  precision=User Defined  arith_type="Signed  (2's comp)"  n_bits=16  bin_pt=15  quantization="Round  (unbiased: +/- Inf)"  overflow=Flag as error  XmcBlockStatus=1  maskContainerNames=group2  block_type=shift  block_config=sysgen:Shift_config
  Shift2 : hdlBasic/Shift  shift_dir=Left  shift_bits=6  en=off  latency=0  precision=User Defined  arith_type="Signed  (2's comp)"  n_bits=16  bin_pt=15  quantization="Round  (unbiased: +/- Inf)"  overflow=Flag as error  XmcBlockStatus=1  maskContainerNames=group2  block_type=shift  block_config=sysgen:Shift_config
  valid : Outport
  rr : Outport  Port=2
  ii : Outport  Port=3
  wires:
  r/1 -> Inverse FFT/1
  i/1 -> Inverse FFT/2
  en/1 -> Inverse FFT/3
  Inverse FFT/1 -> Register5/1
  Inverse FFT/2 -> Register1/1
  Constant1/1 -> Register2/1
  Inverse FFT/3 -> Register2/2
  Register2/1 -> valid/1
  Register5/1 -> Shift2/1
  Register1/1 -> Shift1/1
  Shift2/1 -> rr/1
  Shift1/1 -> ii/1

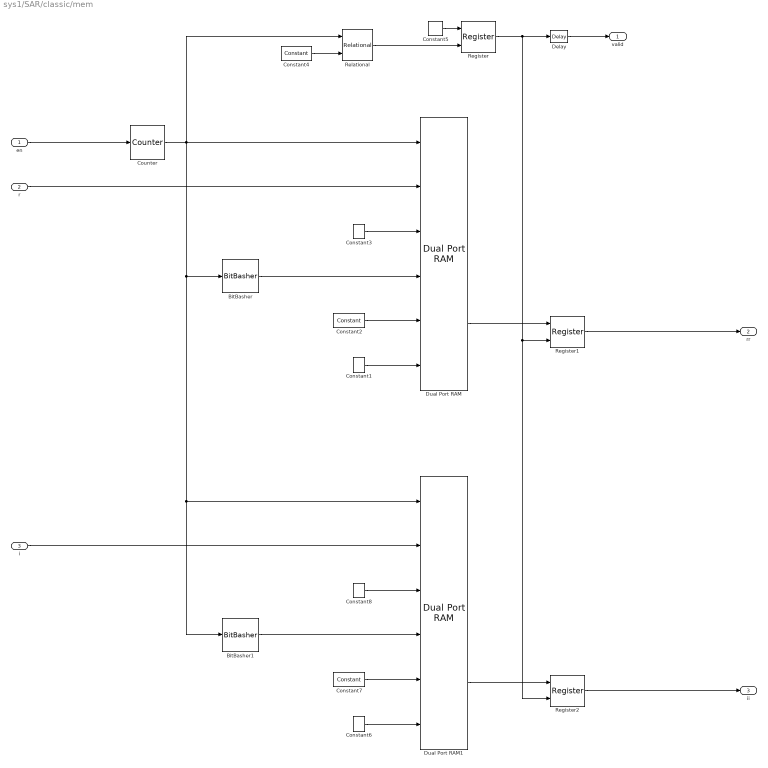
== system sys1/SAR/classic/mem ==
  en : Inport
  r : Inport  Port=2
  i : Inport  Port=3
  BitBasher : hdlBasic/BitBasher  bitexpr=ab={a[19],a[8:0],a[18:9]}  display_expr=off  sr_1=ab  arith_type1=Unsigned  bin_pt1=0  sr_2=2  arith_type2=Unsigned  bin_pt2=0  sr_3=3  arith_type3=Unsigned  bin_pt3=0  sr_4=4  arith_type4=Unsigned  bin_pt4=0  XmcBlockStatus=1  maskContainerNames=group1  block_type=bitbasher  block_config=sysgen:BitBasher_config
  BitBasher1 : hdlBasic/BitBasher  bitexpr=ab={a[19],a[8:0],a[18:9]}  display_expr=off  sr_1=ab  arith_type1=Unsigned  bin_pt1=0  sr_2=2  arith_type2=Unsigned  bin_pt2=0  sr_3=3  arith_type3=Unsigned  bin_pt3=0  sr_4=4  arith_type4=Unsigned  bin_pt4=0  XmcBlockStatus=1  maskContainerNames=group1  block_type=bitbasher  block_config=sysgen:BitBasher_config
  Constant1 : hdlBasic/Constant  const=0  gui_display_data_type=Boolean  arith_type=Boolean  n_bits=16  bin_pt=14  preci_type=Single  exp_width=8  frac_width=24  explicit_period=on  period=ts  XmcBlockStatus=1  maskContainerNames=tabcontainer1  block_type=constant  block_config=sysgen:Constant_config
  Constant2 : hdlBasic/Constant  const=0  gui_display_data_type=Fixed-point  arith_type=Signed (2's comp)  n_bits=16  bin_pt=15  preci_type=Single  exp_width=8  frac_width=24  explicit_period=on  period=ts  XmcBlockStatus=1  maskContainerNames=tabcontainer1  block_type=constant  block_config=sysgen:Constant_config
  Constant3 : hdlBasic/Constant  const=1  gui_display_data_type=Boolean  arith_type=Boolean  n_bits=16  bin_pt=14  preci_type=Single  exp_width=8  frac_width=24  explicit_period=on  period=ts  XmcBlockStatus=1  maskContainerNames=tabcontainer1  block_type=constant  block_config=sysgen:Constant_config
  Constant4 : hdlBasic/Constant  const=2^20-1  gui_display_data_type=Fixed-point  arith_type=Unsigned  n_bits=20  bin_pt=0  preci_type=Single  exp_width=8  frac_width=24  explicit_period=on  period=ts  XmcBlockStatus=1  maskContainerNames=tabcontainer1  block_type=constant  block_config=sysgen:Constant_config
  Constant5 : hdlBasic/Constant  const=1  gui_display_data_type=Boolean  arith_type=Boolean  n_bits=20  bin_pt=0  preci_type=Single  exp_width=8  frac_width=24  explicit_period=on  period=ts  XmcBlockStatus=1  maskContainerNames=tabcontainer1  block_type=constant  block_config=sysgen:Constant_config
  Constant6 : hdlBasic/Constant  const=0  gui_display_data_type=Boolean  arith_type=Boolean  n_bits=16  bin_pt=14  preci_type=Single  exp_width=8  frac_width=24  explicit_period=on  period=ts  XmcBlockStatus=1  maskContainerNames=tabcontainer1  block_type=constant  block_config=sysgen:Constant_config
  Constant7 : hdlBasic/Constant  const=0  gui_display_data_type=Fixed-point  arith_type=Signed (2's comp)  n_bits=16  bin_pt=15  preci_type=Single  exp_width=8  frac_width=24  explicit_period=on  period=ts  XmcBlockStatus=1  maskContainerNames=tabcontainer1  block_type=constant  block_config=sysgen:Constant_config
  Constant8 : hdlBasic/Constant  const=1  gui_display_data_type=Boolean  arith_type=Boolean  n_bits=16  bin_pt=14  preci_type=Single  exp_width=8  frac_width=24  explicit_period=on  period=ts  XmcBlockStatus=1  maskContainerNames=tabcontainer1  block_type=constant  block_config=sysgen:Constant_config
  Counter : hdlBasic/Counter  cnt_type=Free running  cnt_to=Inf  operation=Up  start_count=0  cnt_by_val=1  arith_type=Unsigned  n_bits=20  bin_pt=0  load_pin=off  rst=off  en=on  explicit_period=Explicit  period=ts  use_behavioral_HDL=off  implementation=Fabric  XmcBlockStatus=1  maskContainerNames=group1  block_type=counter  block_config=sysgen:Counter_config  block_width=531  block_height=1023
  Delay : hdlBasic/Delay  rst=off  en=off  latency=2  reg_retiming=off  XmcBlockStatus=1  maskContainerNames=group1  block_type=delay  block_config=sysgen:Delay_config
  Dual Port RAM : hdlBasic/Dual Port RAM  depth=2^20  initVector=0  distributed_mem=Block RAM  init_a=0  init_b=0  rst_a=off  rst_b=off  en_a=off  en_b=off  latency=1  write_mode_A=Read After Write  write_mode_B=Read Before Write  explicit_period=[]  period=[]  simulation_type=fast_sim  XmcBlockStatus=1  maskContainerNames=tabcontainer1  block_type=dpram  block_config=sysgen:Dpram_config  optimize=Area
      settings: infoedit=[]
  Dual Port RAM1 : hdlBasic/Dual Port RAM  depth=2^20  initVector=0  distributed_mem=Block RAM  init_a=0  init_b=0  rst_a=off  rst_b=off  en_a=off  en_b=off  latency=1  write_mode_A=Read After Write  write_mode_B=Read Before Write  explicit_period=[]  period=[]  simulation_type=fast_sim  XmcBlockStatus=1  maskContainerNames=tabcontainer1  block_type=dpram  block_config=sysgen:Dpram_config  optimize=Area
      settings: infoedit=[]
  Register : hdlBasic/Register  init=0  rst=off  en=on  XmcBlockStatus=1  maskContainerNames=tabcontainer1  block_type=register  block_config=sysgen:Register_config
  Register1 : hdlBasic/Register  init=0  rst=off  en=on  XmcBlockStatus=1  maskContainerNames=tabcontainer1  block_type=register  block_config=sysgen:Register_config
  Register2 : hdlBasic/Register  init=0  rst=off  en=on  XmcBlockStatus=1  maskContainerNames=tabcontainer1  block_type=register  block_config=sysgen:Register_config
  Relational : hdlBasic/Relational  mode=a=b  op_type=Bool  en=off  latency=0  XmcBlockStatus=1  maskContainerNames=tabcontainer1  block_type=relational  block_config=sysgen:Relational_config
  valid : Outport
  rr : Outport  Port=2
  ii : Outport  Port=3
  wires:
  Constant3/1 -> Dual Port RAM/3
  Constant2/1 -> Dual Port RAM/5
  Constant1/1 -> Dual Port RAM/6
  en/1 -> Counter/1
  r/1 -> Dual Port RAM/2
  BitBasher/1 -> Dual Port RAM/4
  Constant4/1 -> Relational/2
  Relational/1 -> Register/2
  Constant5/1 -> Register/1
  Dual Port RAM/2 -> Register1/1
  Delay/1 -> valid/1
  Dual Port RAM1/2 -> Register2/1
  Register/1 -> Register2/2, Register1/2, Delay/1
  BitBasher1/1 -> Dual Port RAM1/4
  i/1 -> Dual Port RAM1/2
  Constant6/1 -> Dual Port RAM1/6
  Constant7/1 -> Dual Port RAM1/5
  Counter/1 -> Relational/1, BitBasher/1, Dual Port RAM1/1, BitBasher1/1, Dual Port RAM/1
  Constant8/1 -> Dual Port RAM1/3
  Register1/1 -> rr/1
  Register2/1 -> ii/1

== system sys1/SAR/classic/mul ==
  en : Inport
  r : Inport  Port=2
  i : Inport  Port=3
  Complex Multiplier 6.0 : hdlDSPIP/Complex Multiplier 6.0   hasatlast=off  hasatuser=off  atuserwidth=1  hasbtlast=off  hasbtuser=off  btuserwidth=1  multtype=Use_Mults  optimizegoal=Resources  flowcontrol=NonBlocking  outputwidth=32  roundmode=Truncate  hasctrltlast=off  hasctrltuser=off  ctrltuserwidth=1  outtlastbehv=Null  latencyconfig=Automatic  minimumlatency=37  aclken=off  aresetn=off  trim_axipin_name=on  simulation_type=hybrid_sim  simulation_model=sysgen:cmpy_v6_0  data_path_portlist={ 's_axis_a_tdata_real', 's_axis_a_tdata_imag', 's_axis_b_tdata_real', 's_axis_b_tdata_imag', 's_axis_ctrl_tdata_rounding_bit', 'm_axis_dout_tdata_real', 'm_axis_dout_tdata_imag' }  aportwidth=63  bportwidth=63  ip_name=Complex Multiplier  ip_version=6.0  dsptool_ready=true  ipcore_usecache=true  ipcore_useipmodelcache=true  ipcore_verbose=false  ipcore_latency_parameter='minimumlatency'  wrapper_available=true  port_translation_map={ 'aclken' => 'en', 'aresetn' => 'rst'}  XmcBlockStatus=1  maskContainerNames=tabcontainer1  block_type=cmpy_v6_0  block_config=sysgen:rodinimport_config
  Convert1 : hdlBasic/Convert  gui_display_data_type=Fixed-point  arith_type=Signed (2's comp)  n_bits=16  bin_pt=15  float_type=Single  exp_bits=8  fraction_bits=24  quantization="Round  (unbiased: +/- Inf)"  overflow=Saturate  en=off  latency=0  pipeline=off  XmcBlockStatus=1  maskContainerNames=group2  block_type=convert  block_config=sysgen:Convert_config  block_width=595  block_height=885
  Convert2 : hdlBasic/Convert  gui_display_data_type=Fixed-point  arith_type=Signed (2's comp)  n_bits=16  bin_pt=15  float_type=Single  exp_bits=8  fraction_bits=24  quantization="Round  (unbiased: +/- Inf)"  overflow=Saturate  en=off  latency=0  pipeline=off  XmcBlockStatus=1  maskContainerNames=group2  block_type=convert  block_config=sysgen:Convert_config  block_width=595  block_height=885
  Counter1 : hdlBasic/Counter  cnt_type=Free running  cnt_to=Inf  operation=Up  start_count=0  cnt_by_val=1  arith_type=Unsigned  n_bits=19  bin_pt=0  load_pin=off  rst=off  en=on  explicit_period=Explicit  period=ts  use_behavioral_HDL=off  implementation=Fabric  XmcBlockStatus=1  maskContainerNames=group1  block_type=counter  block_config=sysgen:Counter_config  block_width=531  block_height=1023
  Delay{3..5,9..12} (7 alike) : hdlBasic/Delay  rst=off  en=off  latency=1  reg_retiming=off  XmcBlockStatus=1  maskContainerNames=group1  block_type=delay  block_config=sysgen:Delay_config
  ROM1 : hdlBasic/ROM  depth=2^19  initVector=-reshape(imag(H_az1'),1,[])  distributed_mem=Block RAM  rst=off  init_reg=0  en=off  latency=1  gui_display_data_type=Fixed-point  arith_type="Signed  (2's comp)"  n_bits=16  bin_pt=15  preci_type=Single  exp_width=8  frac_width=24  optimize=Area  use_rpm=on  simulation_type=fast_sim  XmcBlockStatus=1  maskContainerNames=tabcontainer1  block_type=sprom  block_config=sysgen:SPROM_config
  ROM2 : hdlBasic/ROM  depth=2^19  initVector=reshape(real(H_az1'),1,[])  distributed_mem=Block RAM  rst=off  init_reg=0  en=off  latency=1  gui_display_data_type=Fixed-point  arith_type="Signed  (2's comp)"  n_bits=16  bin_pt=15  preci_type=Single  exp_width=8  frac_width=24  optimize=Area  use_rpm=on  simulation_type=fast_sim  XmcBlockStatus=1  maskContainerNames=tabcontainer1  block_type=sprom  block_config=sysgen:SPROM_config
  valid : Outport
  rr : Outport  Port=2
  ii : Outport  Port=3
  wires:
  Counter1/1 -> ROM2/1, ROM1/1
  i/1 -> Delay10/1
  r/1 -> Delay11/1
  ROM1/1 -> Complex Multiplier 6.0/5
  Complex Multiplier 6.0/2 -> Convert1/1
  Complex Multiplier 6.0/3 -> Convert2/1
  ROM2/1 -> Complex Multiplier 6.0/6
  en/1 -> Delay9/1, Delay12/1, Counter1/1
  Delay4/1 -> ii/1
  Delay5/1 -> rr/1
  Delay3/1 -> valid/1
  Delay9/1 -> Complex Multiplier 6.0/1
  Delay10/1 -> Complex Multiplier 6.0/2
  Delay11/1 -> Complex Multiplier 6.0/3
  Delay12/1 -> Complex Multiplier 6.0/4
  Complex Multiplier 6.0/1 -> Delay3/1
  Convert1/1 -> Delay4/1
  Convert2/1 -> Delay5/1

== system sys1/SAR/stream/Enabled Subsystem11 ==
  Enable : EnablePort
  Real Channel4 : dspsrcs4/Signal From Workspace  X=real(reshape(xx4,1,[]))*2^-13  Ts=ts  nsamps=1  OutputAfterFinalValue=Cyclic repetition  ignoreOrWarnInputAndFrameLengths=off  OutputFrames=on
  out : Outport
  wires:
  Real Channel4/1 -> out/1

== system sys1/SAR/stream/Enabled Subsystem12 ==
  Enable : EnablePort
  Real Channel4 : dspsrcs4/Signal From Workspace  X=real(reshape(xx5,1,[]))*2^-13  Ts=ts  nsamps=1  OutputAfterFinalValue=Cyclic repetition  ignoreOrWarnInputAndFrameLengths=off  OutputFrames=on
  out : Outport
  wires:
  Real Channel4/1 -> out/1

== system sys1/SAR/stream/Enabled Subsystem13 ==
  Enable : EnablePort
  Real Channel4 : dspsrcs4/Signal From Workspace  X=real(reshape(xx6,1,[]))*2^-22  Ts=ts  nsamps=1  OutputAfterFinalValue=Cyclic repetition  ignoreOrWarnInputAndFrameLengths=off  OutputFrames=on
  out : Outport
  wires:
  Real Channel4/1 -> out/1

== system sys1/SAR/stream/mul ==
  en : Inport
  r : Inport  Port=2
  i : Inport  Port=3
  Complex Multiplier 6.0 : hdlDSPIP/Complex Multiplier 6.0   hasatlast=off  hasatuser=off  atuserwidth=1  hasbtlast=off  hasbtuser=off  btuserwidth=1  multtype=Use_Mults  optimizegoal=Resources  flowcontrol=NonBlocking  outputwidth=32  roundmode=Truncate  hasctrltlast=off  hasctrltuser=off  ctrltuserwidth=1  outtlastbehv=Null  latencyconfig=Automatic  minimumlatency=37  aclken=off  aresetn=off  trim_axipin_name=on  simulation_type=hybrid_sim  simulation_model=sysgen:cmpy_v6_0  data_path_portlist={ 's_axis_a_tdata_real', 's_axis_a_tdata_imag', 's_axis_b_tdata_real', 's_axis_b_tdata_imag', 's_axis_ctrl_tdata_rounding_bit', 'm_axis_dout_tdata_real', 'm_axis_dout_tdata_imag' }  aportwidth=63  bportwidth=63  ip_name=Complex Multiplier  ip_version=6.0  dsptool_ready=true  ipcore_usecache=true  ipcore_useipmodelcache=true  ipcore_verbose=false  ipcore_latency_parameter='minimumlatency'  wrapper_available=true  port_translation_map={ 'aclken' => 'en', 'aresetn' => 'rst'}  XmcBlockStatus=1  maskContainerNames=tabcontainer1  block_type=cmpy_v6_0  block_config=sysgen:rodinimport_config
  Convert1 : hdlBasic/Convert  gui_display_data_type=Fixed-point  arith_type=Signed (2's comp)  n_bits=16  bin_pt=15  float_type=Single  exp_bits=8  fraction_bits=24  quantization="Round  (unbiased: +/- Inf)"  overflow=Saturate  en=off  latency=0  pipeline=off  XmcBlockStatus=1  maskContainerNames=group2  block_type=convert  block_config=sysgen:Convert_config  block_width=595  block_height=885
  Convert2 : hdlBasic/Convert  gui_display_data_type=Fixed-point  arith_type=Signed (2's comp)  n_bits=16  bin_pt=15  float_type=Single  exp_bits=8  fraction_bits=24  quantization="Round  (unbiased: +/- Inf)"  overflow=Saturate  en=off  latency=0  pipeline=off  XmcBlockStatus=1  maskContainerNames=group2  block_type=convert  block_config=sysgen:Convert_config  block_width=595  block_height=885
  Counter1 : hdlBasic/Counter  cnt_type=Free running  cnt_to=Inf  operation=Up  start_count=0  cnt_by_val=1  arith_type=Unsigned  n_bits=19  bin_pt=0  load_pin=off  rst=off  en=on  explicit_period=Explicit  period=ts  use_behavioral_HDL=off  implementation=Fabric  XmcBlockStatus=1  maskContainerNames=group1  block_type=counter  block_config=sysgen:Counter_config  block_width=531  block_height=1023
  Delay{3..5,9..12} (7 alike) : hdlBasic/Delay  rst=off  en=off  latency=1  reg_retiming=off  XmcBlockStatus=1  maskContainerNames=group1  block_type=delay  block_config=sysgen:Delay_config
  ROM1 : hdlBasic/ROM  depth=2^19  initVector=reshape(imag(H_az2),1,[])  distributed_mem=Block RAM  rst=off  init_reg=0  en=off  latency=1  gui_display_data_type=Fixed-point  arith_type="Signed  (2's comp)"  n_bits=16  bin_pt=15  preci_type=Single  exp_width=8  frac_width=24  optimize=Area  use_rpm=on  simulation_type=fast_sim  XmcBlockStatus=1  maskContainerNames=tabcontainer1  block_type=sprom  block_config=sysgen:SPROM_config
  ROM2 : hdlBasic/ROM  depth=2^19  initVector=reshape(real(H_az2),1,[])  distributed_mem=Block RAM  rst=off  init_reg=0  en=off  latency=1  gui_display_data_type=Fixed-point  arith_type="Signed  (2's comp)"  n_bits=16  bin_pt=15  preci_type=Single  exp_width=8  frac_width=24  optimize=Area  use_rpm=on  simulation_type=fast_sim  XmcBlockStatus=1  maskContainerNames=tabcontainer1  block_type=sprom  block_config=sysgen:SPROM_config
  valid : Outport
  rr : Outport  Port=2
  ii : Outport  Port=3
  wires:
  Complex Multiplier 6.0/3 -> Convert2/1
  Complex Multiplier 6.0/2 -> Convert1/1
  Complex Multiplier 6.0/1 -> Delay3/1
  Delay12/1 -> Complex Multiplier 6.0/4
  Delay11/1 -> Complex Multiplier 6.0/3
  Delay10/1 -> Complex Multiplier 6.0/2
  Delay9/1 -> Complex Multiplier 6.0/1
  Delay3/1 -> valid/1
  Delay5/1 -> rr/1
  Delay4/1 -> ii/1
  en/1 -> Delay9/1, Delay12/1, Counter1/1
  ROM2/1 -> Complex Multiplier 6.0/6
  ROM1/1 -> Complex Multiplier 6.0/5
  r/1 -> Delay11/1
  i/1 -> Delay10/1
  Counter1/1 -> ROM1/1, ROM2/1
  Convert1/1 -> Delay4/1
  Convert2/1 -> Delay5/1

== system sys1/SAR/stream/stream_fft ==
  en : Inport
  re : Inport  Port=2
  im : Inport  Port=3
  Scale : hdlBasic/Scale  scale_factor=15  XmcBlockStatus=1  maskContainerNames=group1  block_type=scale  block_config=sysgen:Scale_config
  Scale1 : hdlBasic/Scale  scale_factor=15  XmcBlockStatus=1  maskContainerNames=group1  block_type=scale  block_config=sysgen:Scale_config
  Scale2 : hdlBasic/Scale  scale_factor=-15  XmcBlockStatus=1  maskContainerNames=group1  block_type=scale  block_config=sysgen:Scale_config
  Scale3 : hdlBasic/Scale  scale_factor=-15  XmcBlockStatus=1  maskContainerNames=group1  block_type=scale  block_config=sysgen:Scale_config
  stage1 : Subsystem
  stage2 : Subsystem
  stage3 : Subsystem
  stage4 : Subsystem
  stage5 : Subsystem
  stage6 : Subsystem
  stage7 : Subsystem
  stage8 : Subsystem
  stage9 : Subsystem
  valid : Outport
  out re : Outport  Port=2
  out im : Outport  Port=3
  wires:
  stage9/3(out_im) -> stage8/3(im)
  en/1 -> stage9/1(en)
  stage9/1(valid) -> stage8/1(en)
  re/1 -> Scale/1
  im/1 -> Scale1/1
  stage9/2(out_re) -> stage8/2(re)
  stage8/3(out_im) -> stage7/3(im)
  stage8/2(out_re) -> stage7/2(re)
  stage8/1(valid) -> stage7/1(en)
  stage7/1(valid) -> stage6/1(en)
  stage7/2(out_re) -> stage6/2(re)
  stage7/3(out_im) -> stage6/3(im)
  stage6/3(out_im) -> stage5/3(im)
  stage6/2(out_re) -> stage5/2(re)
  stage6/1(valid) -> stage5/1(en)
  stage5/1(valid) -> stage4/1(en)
  stage5/2(out_re) -> stage4/2(re)
  stage5/3(out_im) -> stage4/3(im)
  stage4/3(out_im) -> stage3/3(im)
  stage4/2(out_re) -> stage3/2(re)
  stage4/1(valid) -> stage3/1(en)
  stage3/1(valid) -> stage2/1(en)
  stage3/2(out_re) -> stage2/2(re)
  stage3/3(out_im) -> stage2/3(im)
  stage2/3(out_im) -> stage1/3(im)
  stage2/2(out_re) -> stage1/2(re)
  stage2/1(valid) -> stage1/1(en)
  stage1/1(valid) -> valid/1
  stage1/2(out_re) -> Scale2/1
  stage1/3(out_im) -> Scale3/1
  Scale/1 -> stage9/2(re)
  Scale1/1 -> stage9/3(im)
  Scale2/1 -> out re/1
  Scale3/1 -> out im/1
